simulink model "simulink_model_non_linear"  (R2026b)
settings: Solver=VariableStepAuto
values from neighbouring files (symbols this model uses):
  Iz = 1960    [Vehicle_Params.m]
  lf = 1.177    [Vehicle_Params.m]
  lr = 1.358    [Vehicle_Params.m]
  m = 1400    [Vehicle_Params.m]
  udry = [1.11, 23.99, 0.52]    [Vehicle_Params.m]
  v = 1    [Vehicle_Params.m]
undefined symbols (not defined in the file or in its folder): Alpha_f_calculate, Alpha_r_calculate, Fd_calculate_linear, Fx_calculate_non_linear, Fy_calculate_non_linear, lambda_calculate
settings Model: Creator=osganig  LastModifiedBy=manel
settings RTWCC: GPUComputeCapability=5.0

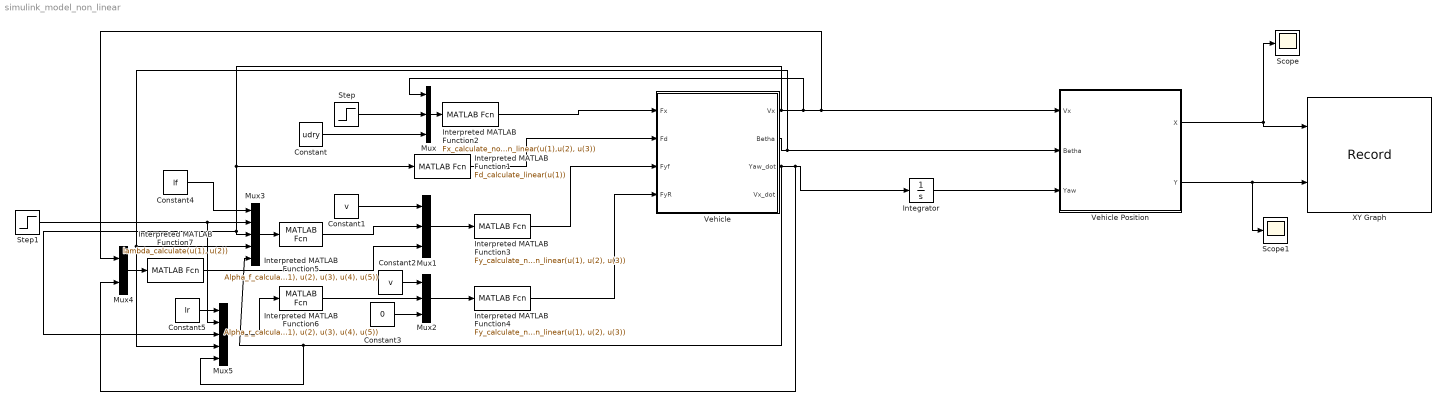
== system simulink_model_non_linear ==
  Constant : Constant  Value=udry
  Constant1 : Constant  Value=v
  Constant2 : Constant  Value=v
  Constant3 : Constant  Value=0
  Constant4 : Constant  Value=lf
  Constant5 : Constant  Value=lr
  Integrator : Integrator
  Interpreted MATLAB Function1 : MATLABFcn  MATLABFcn=Fd_calculate_linear(u(1))
  Interpreted MATLAB Function2 : MATLABFcn  MATLABFcn=Fx_calculate_non_linear(u(1),u(2), u(3))
  Interpreted MATLAB Function3 : MATLABFcn  MATLABFcn=Fy_calculate_non_linear(u(1), u(2), u(3))
  Interpreted MATLAB Function4 : MATLABFcn  MATLABFcn=Fy_calculate_non_linear(u(1), u(2), u(3))
  Interpreted MATLAB Function5 : MATLABFcn  MATLABFcn=Alpha_f_calculate(u(1), u(2), u(3), u(4), u(5))
  Interpreted MATLAB Function6 : MATLABFcn  MATLABFcn=Alpha_r_calculate(u(1), u(2), u(3), u(4), u(5))
  Interpreted MATLAB Function7 : MATLABFcn  MATLABFcn=lambda_calculate(u(1), u(2))
  Mux : Mux  Inputs=3
  Mux1 : Mux  Inputs=3
  Mux2 : Mux  Inputs=3
  Mux3 : Mux  Inputs=5
  Mux4 : Mux  Inputs=2
  Mux5 : Mux  Inputs=5
  Scope : Scope
  Scope1 : Scope
  Step : Step  FinalValue=w_input  SampleTime=0
  Step1 : Step  FinalValue=delta_input  SampleTime=0
  Vehicle : Subsystem
  Vehicle Position : Subsystem
  XY Graph : Record  NumPorts=2.0  FileSettingsInternal="{\"entries\":[{\"content\":{\"excelSettings\":{\"content\":{},\"type\":\"Streamout.ExcelSettings\"},\"parquetSettings\":{\"content\":{},\"type\":\"Streamout.ParquetSettings\"}},\"type\":\"Streamout.FileSettingStorage\",\"uuid\":\"\"}],\"packageUris\":[\"http:\\/\\/schema.mathworks.com\\/mf0\\/streamout_blocks\\/R2020a\"],\"version\":\"1.0\"}"  FrameSettings=[0, 0]  Layout=[1 1]  SignalsInternal="{\"entries\":[{\"content\":{\"signals\":[{\"content\":{\"blockPath\":[],\"dimensions\":[1],\"domain\":\"\",\"lineColor\":\"#a2142f\",\"plots\":[ 1 ],\"port\":1,\"sid\":[\"\"],\"signalID\":1,\"signalName\":\"Vehicle Position:1\"},\"type\":\"RecordBlkView.Signal\",\"uuid\":\"\"},{\"content\":{\"blockPath\":[],\"dimensions\":[1],\"domain\":\"\",\"lineColor\":\"#139fff\",\"plots\":[ 1 ],\"port\":2,\"sid\":[\"\"],\"signalID\":2,\"signalName\":\"Vehicle Position:2\"},\"type\":\"RecordBlkView.Signal\",\"uuid\":\"\"}]},\"type\":\"RecordBlkView.InputSignals\",\"uuid\":\"\"}],\"packageUris\":[\"http:\\/\\/schema.mathworks.com\\/mf0\\/streamout_blocks\\/R2020a\"],\"version\":\"1.0\"}"  VisualizationBindings="{\"xyplotplugin\":{\"info\":[{\"series\":[{\"bindingParametersList\":[{\"parameter\":\"X-Axis\",\"signalID\":1,\"signalName\":\"Vehicle Position:1\"},{\"parameter\":\"Y-Axis\",\"signalID\":2,\"signalName\":\"Vehicle Position:2\"}],\"seriesID\":0}],\"subplotID\":1}]}}"  CompatibilityTag=XY
  wires:
  Interpreted MATLAB Function3/1 -> Vehicle/3(Fyf)
  Interpreted MATLAB Function4/1 -> Vehicle/4(FyR)
  Interpreted MATLAB Function1/1 -> Vehicle/2(Fd)
  Vehicle/2(Betha) -> Mux5/4, Mux3/4, Vehicle Position/2(Betha)
  Vehicle/3(Yaw_dot) -> Mux5/5, Mux3/5, Mux4/2, Integrator/1
  Integrator/1 -> Vehicle Position/3(Yaw)
  Vehicle Position/1(X) -> Scope/1, XY Graph/1
  Vehicle Position/2(Y) -> Scope1/1, XY Graph/2
  Interpreted MATLAB Function2/1 -> Vehicle/1(Fx)
  Mux1/1 -> Interpreted MATLAB Function3/1
  Mux2/1 -> Interpreted MATLAB Function4/1
  Step/1 -> Mux/2
  Step1/1 -> Mux5/2, Mux3/2
  Constant/1 -> Mux/3
  Interpreted MATLAB Function5/1 -> Mux1/2
  Interpreted MATLAB Function6/1 -> Mux2/2
  Mux3/1 -> Interpreted MATLAB Function5/1
  Vehicle/1(Vx) -> Mux/1, Mux4/1, Vehicle Position/1(Vx), Mux5/3, Mux3/3, Interpreted MATLAB Function1/1
  Constant1/1 -> Mux1/1
  Interpreted MATLAB Function7/1 -> Mux1/3
  Mux4/1 -> Interpreted MATLAB Function7/1
  Constant2/1 -> Mux2/1
  Constant3/1 -> Mux2/3
  Constant4/1 -> Mux3/1
  Mux5/1 -> Interpreted MATLAB Function6/1
  Constant5/1 -> Mux5/1
  Mux/1 -> Interpreted MATLAB Function2/1

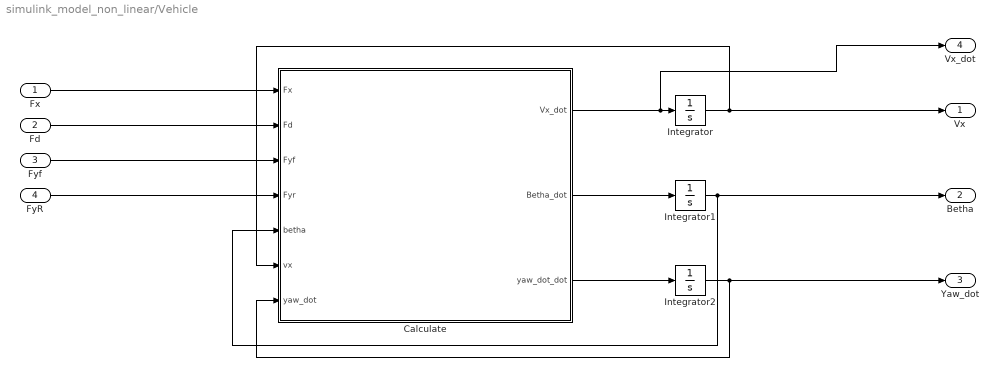
== system simulink_model_non_linear/Vehicle ==
  Fx : Inport
  Fd : Inport  Port=2
  Fyf : Inport  Port=3
  FyR : Inport  Port=4
  "Calculate " : MATLAB Function  TreatAsAtomicUnit=on
  Integrator : Integrator
  Integrator1 : Integrator
  Integrator2 : Integrator
  Vx : Outport
  Betha : Outport  Port=2
  Yaw_dot : Outport  Port=3
  Vx_dot : Outport  Port=4
  wires:
  Fx/1 -> "Calculate "/1(Fx)
  Fd/1 -> "Calculate "/2(Fd)
  Fyf/1 -> "Calculate "/3(Fyf)
  FyR/1 -> "Calculate "/4(Fyr)
  "Calculate "/1(Vx_dot) -> Vx_dot/1, Integrator/1
  "Calculate "/2(Betha_dot) -> Integrator1/1
  "Calculate "/3(yaw_dot_dot) -> Integrator2/1
  Integrator2/1 -> Yaw_dot/1, "Calculate "/7(yaw_dot)
  Integrator1/1 -> Betha/1, "Calculate "/5(betha)
  Integrator/1 -> Vx/1, "Calculate "/6(vx)

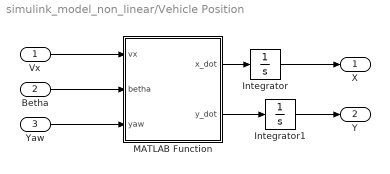
== system simulink_model_non_linear/Vehicle Position ==
  Vx : Inport
  Betha : Inport  Port=2
  Yaw : Inport  Port=3
  Integrator : Integrator
  Integrator1 : Integrator
  MATLAB Function : MATLAB Function  TreatAsAtomicUnit=on
  X : Outport
  Y : Outport  Port=2
  wires:
  Vx/1 -> MATLAB Function/1(vx)
  Betha/1 -> MATLAB Function/2(betha)
  Yaw/1 -> MATLAB Function/3(yaw)
  MATLAB Function/1(x_dot) -> Integrator/1
  Integrator/1 -> X/1
  MATLAB Function/2(y_dot) -> Integrator1/1
  Integrator1/1 -> Y/1

== matlab function simulink_model_non_linear/Vehicle/Calculate  ==
  data: Fx input; Vx_dot output; Fd input; Fyf input; Fyr input; betha input; vx input; yaw_dot input; Betha_dot output; yaw_dot_dot output; m parameter; Iz parameter; lf parameter; lr parameter
function [Vx_dot,Betha_dot,yaw_dot_dot]= fcn(Fx,Fd,Fyf,Fyr,betha,vx,yaw_dot, m, Iz, lf, lr)

Vx_dot = (1/m )*(Fx - Fd) + betha*vx*yaw_dot;
Betha_dot = (1/(m*max(vx,0.1)))*(Fyf + Fyr) - yaw_dot;
yaw_dot_dot = (1/Iz) * (Fyf * lf - Fyr* lr);

== matlab function simulink_model_non_linear/Vehicle Position/MATLAB Function ==
  data: vx input; betha input; x_dot output; yaw input; y_dot output
function [x_dot,y_dot] = fcn(vx,betha,yaw)

vy = vx* tan(betha);
x_dot = vx*cos(yaw) - vy*sin(yaw);
y_dot = vx*sin(yaw) - vy*cos(yaw);
